simulink model "ECG_Rhythm_PVC_Detection_PaperArchitecture"  (R2019a)
settings: Solver=FixedStepDiscrete  StartTime=0.0  StopTime=10  FixedStep=1/360  RelTol=1e-3
libraries: simulink x14, dspstat3 x5, dspfdesign x2
settings Model: Creator=atif  LastModifiedBy=Admin
settings HardwareCC: ProdHWDeviceType=AMD->x86-64 (Windows64)

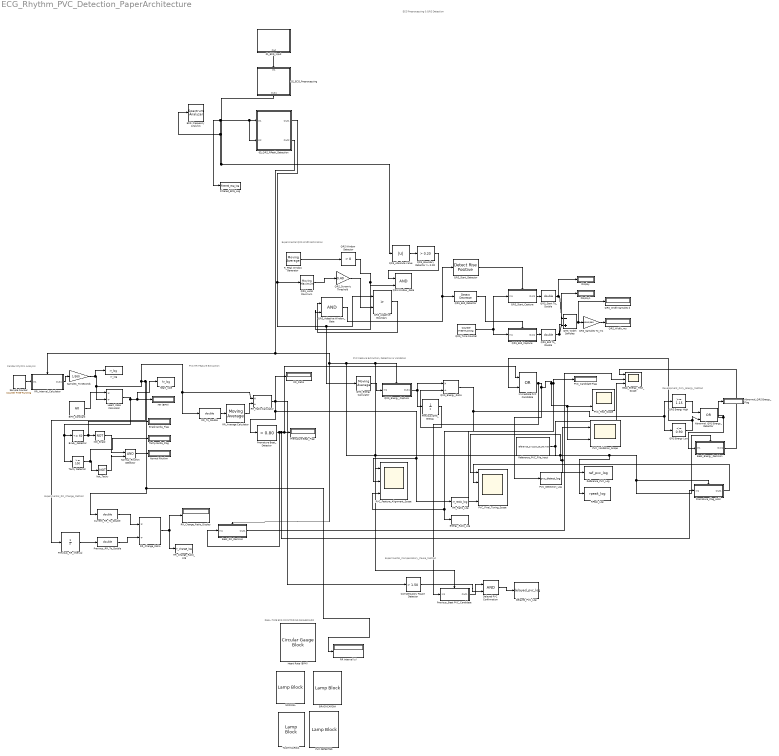
== system ECG_Rhythm_PVC_Detection_PaperArchitecture ==
  note: REAL-TIME ECG MONITORING DASHBOARD
  note: Development_Only_Energy_Method
  note: Experimental_Compensatory_Pause_Method
  note: PVC Feature Extraction, Detection & Validation
  note: Experimental_RR_Change_Method
  note: Experimental QRS Width Estimation
  note: PVC RR Feature Extraction
  note: Cardiac Rhythm Analysis
  note: ECG Preprocessing & QRS Detection
  01_ECG_Input : Subsystem
  02_ECG_Preprocessing : Subsystem
  03_QRS_RPeak_Detection : Subsystem
  Abnormal_QRS Energy_Detector : Logic  Operator=OR  IconShape=distinctive  AllPortsSameDT=off  OutDataTypeStr=boolean
  Abnormal_QRS Energy_Flag : Display
  BPM_Constant : Constant  Value=60
  BRADYCARDIA : LampBlock  LabelPosition=Hide
  Beat_Energy_Decision : Subsystem  TreatAsAtomicUnit=on
  Beat_Energy_Test_Scope : Scope  NumInputPorts=3
  Beat_RR_Decision : Subsystem  TreatAsAtomicUnit=on
  Brady_Detector : simulink/Logic and Bit Operations/Compare To Constant  relop=<=  const=60  OutDataTypeStr=boolean
  Bradycardia_Flag : Display
  Compensatory Pause Detector : simulink/Logic and Bit Operations/Compare To Constant  relop=>  const=1.50  OutDataTypeStr=boolean
  Current_RR_To_Double : DataTypeConversion  OutDataTypeStr=double
  "Delayed PVC Confirmation " : Logic  IconShape=distinctive  AllPortsSameDT=off  OutDataTypeStr=boolean
  Delayed_PVC_Log : ToWorkspace  VariableName=delayed_pvc_log  SaveFormat=Structure With Time  SampleTime=-1
  Display : Display
  Display1 : Display
  ECG_Frequency Analysis : SpectrumAnalyzer
  Energy_Ratio_Log : ToWorkspace  VariableName=energy_ratio_log  SaveFormat=Structure With Time  SampleTime=-1
  Filtered_ECG_Log : ToWorkspace  VariableName=filtered_ecg_log  SaveFormat=Structure With Time  SampleTime=-1
  HR (BPM) : Display
  Heart Rate (BPM) : CircularGaugeBlock  Tag=Heart Rate (BPM)  LabelPosition=Hide  ScaleMin=40  ScaleMax=140
  Heart_Rate Calculator : Product  Inputs=*/
  "Immediate PVC Candidate " : Logic  Operator=OR  AllPortsSameDT=off  OutDataTypeStr=boolean
  NORMAL : LampBlock  LabelPosition=Hide
  Normal Rhythm : Display
  Normal_Rhythm Detector : Logic  IconShape=distinctive  AllPortsSameDT=off  OutDataTypeStr=boolean
  Not_Brady : Logic  Operator=NOT  IconShape=distinctive  AllPortsSameDT=off  OutDataTypeStr=boolean
  Not_Tachy : Logic  Operator=NOT  IconShape=distinctive  AllPortsSameDT=off  OutDataTypeStr=boolean
  PVC DETECTED : LampBlock  LabelPosition=Hide
  PVC_Candidate Flag : Display
  PVC_Detection_Log : ToWorkspace  VariableName=pvc_detect_log  SaveFormat=Structure With Time  SampleTime=-1
  PVC_Feature_Alignment_Scope : Scope  NumInputPorts=3
  PVC_Final_Tuning_Scope : Scope  NumInputPorts=4
  PVC_Test_Scope : Scope  NumInputPorts=3
  PVC_Validation_Scope : Scope  NumInputPorts=2
  Premature Beat_Detector : simulink/Logic and Bit Operations/Compare To Constant  relop=<  const=0.80  OutDataTypeStr=boolean
  Premature Beat_Flag : Display
  Premature_Flag_Hold : Subsystem  TreatAsAtomicUnit=on
  Previous QRS_Energy : UnitDelay  SampleTime=-1  HasFrameUpgradeWarning=on
  Previous_Beat PVC_Candidate : Subsystem  TreatAsAtomicUnit=on
  Previous_RR_Interval : UnitDelay  SampleTime=-1  HasFrameUpgradeWarning=on
  Previous_RR_To_Double : DataTypeConversion  OutDataTypeStr=double
  QRS Energy High : simulink/Logic and Bit Operations/Compare To Constant  relop=>=  const=1.15  OutDataTypeStr=boolean
  QRS Energy Low : simulink/Logic and Bit Operations/Compare To Constant  relop=<=  const=0.90  OutDataTypeStr=boolean
  QRS Window Detector : simulink/Logic and Bit Operations/Compare To Constant  relop=>  const=0  OutDataTypeStr=boolean
  QRS Window_Gate : Logic  IconShape=distinctive  AllPortsSameDT=off  OutDataTypeStr=boolean
  QRS_Absolute Value : Abs
  QRS_Adaptive Boundary : RelationalOperator  Operator=>  OutDataTypeStr=boolean  RndMeth=Simplest
  QRS_Adaptive Window_Gate : Logic  IconShape=distinctive  AllPortsSameDT=off  OutDataTypeStr=boolean
  QRS_Boundary Detector (> 0.20) : simulink/Logic and Bit Operations/Compare To Constant  relop=>  const=0.20  OutDataTypeStr=boolean
  "QRS_Dynamic Threshold " : Gain  Gain=0.40
  QRS_End To_Double : DataTypeConversion  OutDataTypeStr=double
  QRS_End_Capture : Subsystem  TreatAsAtomicUnit=on
  QRS_End_Detector : simulink/Logic and Bit Operations/Detect Decrease  vinit=0.0  OutDataTypeStr=boolean
  QRS_Energy Calculator : dspstat3/Moving Average  Method=Sliding window  ForgettingFactorPort=off  SpecifyWindowLength=on  WindowLength=54  ForgettingFactor=0.9  SimulateUsing=Code generation
  QRS_Energy_Capture : Subsystem  TreatAsAtomicUnit=on
  "QRS_Energy_Ratio " : Product  Inputs=*/
  QRS_Local Maximum : dspstat3/Moving Maximum  SpecifyWindowLength=on  WindowLength=36  SimulateUsing=Code generation
      settings: SourceProductName=DSP System Toolbox  SourceProductBaseCode=DS
  QRS_Samples To_ms : Gain  Gain=1000/360
  QRS_Start To_Double : DataTypeConversion  OutDataTypeStr=double
  QRS_Start_Capture : Subsystem  TreatAsAtomicUnit=on
  QRS_Start_Detector : simulink/Logic and Bit Operations/Detect Rise Positive  vinit=0  OutDataTypeStr=boolean
  QRS_Time Counter : simulink/Sources/Counter Free-Running  NumBits=32  tsamp=1/360
  QRS_Width Samples : Sum  Inputs=-+
  QRS_Width Samples d : Display
  QRS_Width_ms : Display
  RPeak_Log : ToWorkspace  VariableName=rpeak_log  SaveFormat=Structure With Time  SampleTime=-1
  RR Interval (s) : Display
  RR_Average Calculator : dspstat3/Moving Average  Method=Sliding window  ForgettingFactorPort=off  SpecifyWindowLength=on  WindowLength=8  ForgettingFactor=0.9  SimulateUsing=Code generation
  RR_Change_Ratio : Product  Inputs=*/
  RR_Change_Ratio_Display : Display
  RR_Change_Ratio_Log : ToWorkspace  VariableName=rr_change_log  SaveFormat=Structure With Time  SampleTime=-1
  RR_Interval_Calculator : Subsystem  TreatAsAtomicUnit=on
  RR_Ratio : Display
  RR_Ratio Calculator : Product  Inputs=*/
  RR_Ratio_Log : ToWorkspace  VariableName=rr_ratio_log  SaveFormat=Structure With Time  SampleTime=-1
  RR_To_Double : DataTypeConversion  OutDataTypeStr=double
  R_Peak Window Generator : dspstat3/Moving Average  Method=Sliding window  ForgettingFactorPort=off  SpecifyWindowLength=on  WindowLength=54  ForgettingFactor=0.9  SimulateUsing=Code generation
  Reference_PVC_File_Input : FromFile  FileName=reference_pvc119_20_30.mat  SampleTime=0
  Reference_PVC_Log : ToWorkspace  VariableName=ref_pvc_log  SaveFormat=Structure With Time  SampleTime=-1
  Sample Counter : simulink/Sources/Counter Free-Running  NumBits=32  tsamp=1/360
  Samples_To Seconds : Gain  Gain=1/360
  TACHYCARDIA : LampBlock  LabelPosition=Hide
  Tachy Detector : simulink/Logic and Bit Operations/Compare To Constant  relop=>=  const=100  OutDataTypeStr=boolean
  Tachycardia_Flag : Display
  heart_rate : ToWorkspace  VariableName=hr_log  SaveFormat=Structure With Time  SampleTime=-1
  rr_log : ToWorkspace  VariableName=rr_log  SaveFormat=Structure With Time  SampleTime=-1
  wires:
  Sample Counter/1 -> RR_Interval_Calculator/1(In1)
  RR_Interval_Calculator/1(Out1) -> Samples_To Seconds/1
  Samples_To Seconds/1 -> rr_log/1, RR_To_Double/1, RR_Ratio Calculator/1, Previous_RR_Interval/1, Current_RR_To_Double/1, RR Interval (s)/1, Heart_Rate Calculator/2
  BPM_Constant/1 -> Heart_Rate Calculator/1
  Heart_Rate Calculator/1 -> Tachy Detector/1, Brady_Detector/1, heart_rate/1, HR (BPM)/1
  Brady_Detector/1 -> Bradycardia_Flag/1, Not_Brady/1
  Tachy Detector/1 -> Not_Tachy/1, Tachycardia_Flag/1
  Not_Tachy/1 -> Normal_Rhythm Detector/2
  Not_Brady/1 -> Normal_Rhythm Detector/1
  Normal_Rhythm Detector/1 -> Normal Rhythm/1
  RR_Average Calculator/1 -> RR_Ratio Calculator/2
  RR_Ratio Calculator/1 -> Compensatory Pause Detector/1, RR_Ratio_Log/1, PVC_Feature_Alignment_Scope/2, Premature Beat_Detector/1, RR_Ratio/1
  RR_To_Double/1 -> RR_Average Calculator/1
  Premature Beat_Detector/1 -> Beat_RR_Decision/1(In1), Premature_Flag_Hold/1(In1), "Immediate PVC Candidate "/1, Premature Beat_Flag/1
  QRS_Absolute Value/1 -> QRS_Boundary Detector (> 0.20)/1
  QRS_Boundary Detector (> 0.20)/1 -> QRS Window_Gate/1
  QRS_Start_Detector/1 -> QRS_Start_Capture/Trigger
  QRS_Time Counter/1 -> QRS_End_Capture/1(In1), QRS_Start_Capture/1(In1)
  QRS_End_Detector/1 -> QRS_End_Capture/Trigger
  QRS_Start_Capture/1(Out1) -> QRS_Start To_Double/1
  QRS_Start To_Double/1 -> Display/1, QRS_Width Samples/1
  QRS_End_Capture/1(Out1) -> QRS_End To_Double/1
  QRS_End To_Double/1 -> Display1/1, QRS_Width Samples/2
  QRS_Width Samples/1 -> QRS_Width Samples d/1, QRS_Samples To_ms/1
  QRS_Samples To_ms/1 -> QRS_Width_ms/1
  R_Peak Window Generator/1 -> QRS Window Detector/1
  QRS Window Detector/1 -> QRS_Adaptive Window_Gate/2, QRS Window_Gate/2
  QRS_Local Maximum/1 -> "QRS_Dynamic Threshold "/1
  "QRS_Dynamic Threshold "/1 -> QRS_Adaptive Boundary/2
  QRS_Adaptive Boundary/1 -> QRS_Adaptive Window_Gate/1
  QRS_Adaptive Window_Gate/1 -> QRS_End_Detector/1, QRS_Start_Detector/1
  QRS_Energy Calculator/1 -> QRS_Energy_Capture/1(In1)
  QRS_Energy_Capture/1(Out1) -> "QRS_Energy_Ratio "/1, Previous QRS_Energy/1
  Previous QRS_Energy/1 -> "QRS_Energy_Ratio "/2
  "QRS_Energy_Ratio "/1 -> Energy_Ratio_Log/1, PVC_Feature_Alignment_Scope/3, QRS Energy Low/1, QRS Energy High/1
  QRS Energy High/1 -> Abnormal_QRS Energy_Detector/1
  QRS Energy Low/1 -> "Immediate PVC Candidate "/2, Abnormal_QRS Energy_Detector/2
  Abnormal_QRS Energy_Detector/1 -> Beat_Energy_Decision/1(In1), Abnormal_QRS Energy_Flag/1
  "Immediate PVC Candidate "/1 -> Previous_Beat PVC_Candidate/1(In1), PVC_Detection_Log/1, PVC_Validation_Scope/2, PVC_Test_Scope/3, PVC_Candidate Flag/1, PVC_Final_Tuning_Scope/4
  Premature_Flag_Hold/1(Out1) -> PVC_Final_Tuning_Scope/2
  Reference_PVC_File_Input/1 -> Reference_PVC_Log/1, PVC_Validation_Scope/1, PVC_Final_Tuning_Scope/1, Beat_Energy_Test_Scope/3
  Beat_Energy_Decision/1(Out1) -> Beat_Energy_Test_Scope/1
  Beat_RR_Decision/1(Out1) -> Beat_Energy_Test_Scope/2
  Previous_RR_Interval/1 -> Previous_RR_To_Double/1
  RR_Change_Ratio/1 -> RR_Change_Ratio_Display/1, RR_Change_Ratio_Log/1
  Current_RR_To_Double/1 -> RR_Change_Ratio/1
  Previous_RR_To_Double/1 -> RR_Change_Ratio/2
  Previous_Beat PVC_Candidate/1(Out1) -> "Delayed PVC Confirmation "/1
  Compensatory Pause Detector/1 -> "Delayed PVC Confirmation "/2
  "Delayed PVC Confirmation "/1 -> Delayed_PVC_Log/1
  02_ECG_Preprocessing/1(Out1) -> 03_QRS_RPeak_Detection/2(In2), 03_QRS_RPeak_Detection/1(In1), Filtered_ECG_Log/1, ECG_Frequency Analysis/1, QRS_Absolute Value/1
  01_ECG_Input/1(Out) -> 02_ECG_Preprocessing/1(In1)
  03_QRS_RPeak_Detection/2(Out2) -> RR_Interval_Calculator/Trigger, QRS_Energy_Capture/Trigger, Previous_Beat PVC_Candidate/Trigger, Beat_Energy_Decision/Trigger, Premature_Flag_Hold/Trigger, RPeak_Log/1, PVC_Feature_Alignment_Scope/1, Beat_RR_Decision/Trigger
  03_QRS_RPeak_Detection/1(Out1) -> QRS_Adaptive Boundary/1, QRS_Energy Calculator/1, QRS_Local Maximum/1

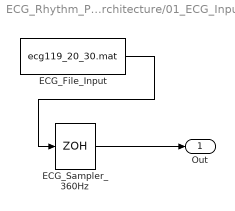
== system ECG_Rhythm_PVC_Detection_PaperArchitecture/01_ECG_Input ==
  "ECG_File_Input " : FromFile  FileName=ecg119_20_30.mat  SampleTime=0
  ECG_Sampler_360Hz : ZeroOrderHold  SampleTime=1/360
  Out : Outport
  wires:
  "ECG_File_Input "/1 -> ECG_Sampler_360Hz/1
  ECG_Sampler_360Hz/1 -> Out/1

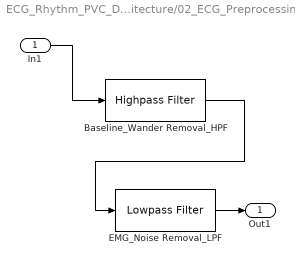
== system ECG_Rhythm_PVC_Detection_PaperArchitecture/02_ECG_Preprocessing ==
  In1 : Inport
  Baseline_Wander Removal_HPF : dspfdesign/Highpass Filter  FilterType=IIR  DesignForMinimumOrder=on  FilterOrder=50  StopbandFrequency=0.1  PassbandFrequency=0.5  StopbandAttenuation=80  PassbandRipple=0.1  InheritSampleRate=off  SampleRate=360  SimulateUsing=Interpreted execution  roundingMode=Floor  coeffsDataTypeStr=fixdt(1,16)
      settings: SourceProductName=DSP System Toolbox
  EMG_Noise Removal_LPF : dspfdesign/Lowpass Filter  FilterType=IIR  DesignForMinimumOrder=on  FilterOrder=50  PassbandFrequency=40  StopbandFrequency=45  PassbandRipple=0.1  StopbandAttenuation=80  InheritSampleRate=off  SampleRate=360  SimulateUsing=Interpreted execution  roundingMode=Floor  coeffsDataTypeStr=fixdt(1,16)
  Out1 : Outport
  wires:
  In1/1 -> Baseline_Wander Removal_HPF/1
  Baseline_Wander Removal_HPF/1 -> EMG_Noise Removal_LPF/1
  EMG_Noise Removal_LPF/1 -> Out1/1

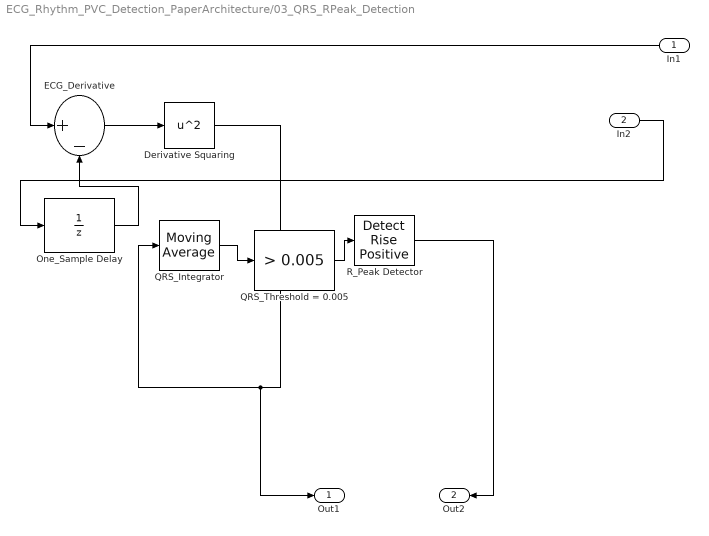
== system ECG_Rhythm_PVC_Detection_PaperArchitecture/03_QRS_RPeak_Detection ==
  In1 : Inport
  In2 : Inport  Port=2
  Derivative Squaring : Math  Operator=square  SaturateOnIntegerOverflow=on
  ECG_Derivative : Sum  Inputs=|+-
  One_Sample Delay : UnitDelay  SampleTime=1/360  HasFrameUpgradeWarning=on
  QRS_Integrator : dspstat3/Moving Average  Method=Sliding window  ForgettingFactorPort=off  SpecifyWindowLength=on  WindowLength=54  ForgettingFactor=0.9  SimulateUsing=Code generation
  QRS_Threshold = 0.005 : simulink/Logic and Bit Operations/Compare To Constant  relop=>  const=0.005  OutDataTypeStr=boolean
  R_Peak Detector : simulink/Logic and Bit Operations/Detect Rise Positive  vinit=0  OutDataTypeStr=boolean
  Out1 : Outport
  Out2 : Outport  Port=2
  wires:
  Derivative Squaring/1 -> Out1/1, QRS_Integrator/1
  QRS_Threshold = 0.005/1 -> R_Peak Detector/1
  ECG_Derivative/1 -> Derivative Squaring/1
  QRS_Integrator/1 -> QRS_Threshold = 0.005/1
  One_Sample Delay/1 -> ECG_Derivative/2
  In2/1 -> One_Sample Delay/1
  In1/1 -> ECG_Derivative/1
  R_Peak Detector/1 -> Out2/1

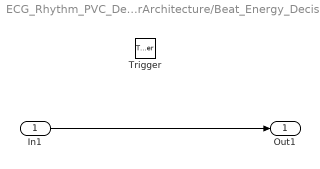
== system ECG_Rhythm_PVC_Detection_PaperArchitecture/Beat_Energy_Decision ==
  In1 : Inport
  Trigger : TriggerPort  VariantControl=Variant
  Out1 : Outport
  wires:
  In1/1 -> Out1/1

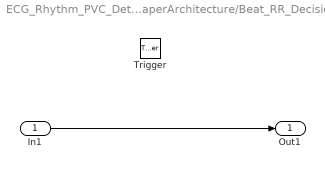
== system ECG_Rhythm_PVC_Detection_PaperArchitecture/Beat_RR_Decision ==
  In1 : Inport
  Trigger : TriggerPort  VariantControl=Variant
  Out1 : Outport
  wires:
  In1/1 -> Out1/1

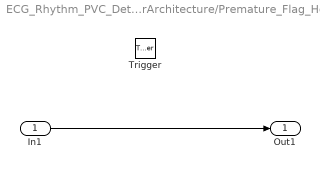
== system ECG_Rhythm_PVC_Detection_PaperArchitecture/Premature_Flag_Hold ==
  In1 : Inport
  Trigger : TriggerPort  VariantControl=Variant
  Out1 : Outport
  wires:
  In1/1 -> Out1/1

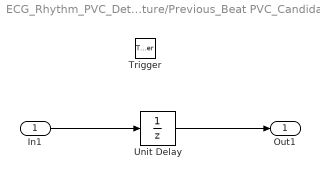
== system ECG_Rhythm_PVC_Detection_PaperArchitecture/Previous_Beat PVC_Candidate ==
  In1 : Inport
  Trigger : TriggerPort  VariantControl=Variant
  Unit Delay : UnitDelay  SampleTime=-1  HasFrameUpgradeWarning=on
  Out1 : Outport
  wires:
  In1/1 -> Unit Delay/1
  Unit Delay/1 -> Out1/1

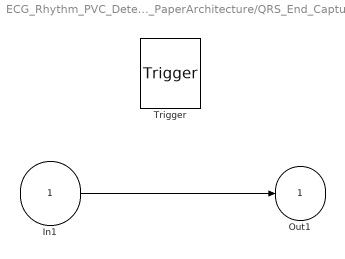
== system ECG_Rhythm_PVC_Detection_PaperArchitecture/QRS_End_Capture ==
  In1 : Inport
  Trigger : TriggerPort  VariantControl=Variant
  Out1 : Outport
  wires:
  In1/1 -> Out1/1

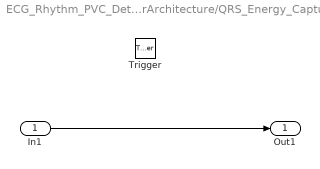
== system ECG_Rhythm_PVC_Detection_PaperArchitecture/QRS_Energy_Capture ==
  In1 : Inport
  Trigger : TriggerPort  VariantControl=Variant
  Out1 : Outport
  wires:
  In1/1 -> Out1/1

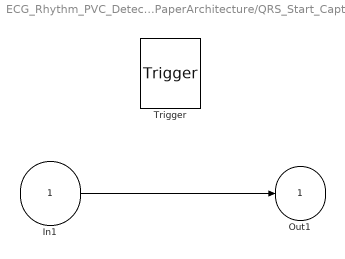
== system ECG_Rhythm_PVC_Detection_PaperArchitecture/QRS_Start_Capture ==
  In1 : Inport
  Trigger : TriggerPort  VariantControl=Variant
  Out1 : Outport
  wires:
  In1/1 -> Out1/1

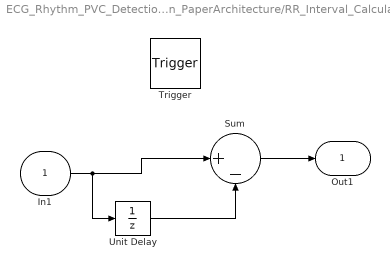
== system ECG_Rhythm_PVC_Detection_PaperArchitecture/RR_Interval_Calculator ==
  In1 : Inport
  Trigger : TriggerPort  VariantControl=Variant
  Sum : Sum  Inputs=|+-
  Unit Delay : UnitDelay  SampleTime=-1  HasFrameUpgradeWarning=on
  Out1 : Outport
  wires:
  In1/1 -> Unit Delay/1, Sum/1
  Unit Delay/1 -> Sum/2
  Sum/1 -> Out1/1
